simulink library "lib_primitives"  (R2026a)
settings: Solver=VariableStepAuto
undefined symbols (not defined in the file or in its folder): Cfi, fref, iC, invL, iR, iTf, L_out, omegab, R_out, Rcf
settings Model: Creator=atomas  LastModifiedBy=atomas

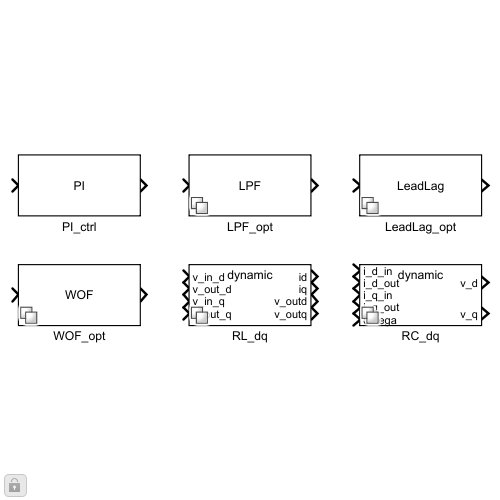
[thumbnail: Simulink's stored preview of the top-level diagram]
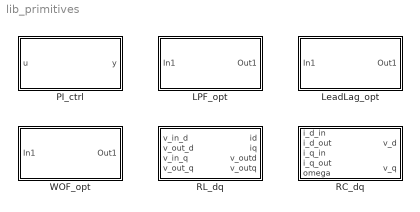
== system lib_primitives ==
  LPF_opt : Subsystem  Variant=on  mask(VFlexP_LPF_opt){T=0.01, x0=0}
      mask prompts: T "Time constant T (0=bypass)"; x0 "Initial state x0"
      mask init:
      | [iTf, use_Tf] = mask_init_opt_filter(T);
      mask Display: disp('LPF')
  LeadLag_opt : Subsystem  Variant=on  mask(VFlexP_LeadLag_opt){Tnum=1, Tden=1, x0=0}
      mask prompts: Tnum "Lead time Tnum"; Tden "Lag time Tden (0=bypass)"; x0 "Initial state x0"
      mask init:
      | [iTf, use_Tf] = mask_init_opt_filter(Tden);
      mask Display: disp('LeadLag')
  PI_ctrl : Subsystem  mask(VFlexP_PI){Kp=1, Ki=1, x0=0}
      mask prompts: Kp "Proportional gain Kp"; Ki "Integral gain Ki"; x0 "Initial condition x0"
      mask Display: disp('PI')
  RC_dq : Subsystem  Variant=on  mask{dynamic=Dynamic, R=Rcf, C=Cfi, fbase=50, x0_d=0, x0_q=0}
      mask prompts: dynamic "Dynamic behavior"; R "Parallel resistance (p.u.)"; C "Capacitance (p.u.)"; fbase "Base frequency (Hz)"; x0_d "Initial v_d"; x0_q "Initial v_q"
      mask init:
      | [iC, iR, omegab, rc_mode] = mask_init_RC(dynamic, R, C, fbase);
      mask TypeOptions dynamic: Dynamic | Static | Static omega
  RL_dq : Subsystem  Variant=on  mask{dynamic=Dynamic, R=R_out, L=L_out, fbase=50, x0_d=0, x0_q=0}
      mask prompts: dynamic "Dynamic behavior"; R "Series resistance (p.u.)"; L "Inductance (p.u.)"; fbase "Base frequency (Hz)"; x0_d "Initial i_d"; x0_q "Initial i_q"
      mask init:
      | [invL, omegab, rl_mode] = mask_init_RL(dynamic, L, fbase);
      mask TypeOptions dynamic: Static | Dynamic | Static omega
  WOF_opt : Subsystem  Variant=on  mask(VFlexP_WOF_opt){K=1, T=1, x0=0}
      mask prompts: K "Gain K"; T "Washout T (0=bypass)"; x0 "Initial state x0"
      mask init:
      | [iTf, use_Tf] = mask_init_opt_filter(T); if all(K == 0), use_Tf = 0; end
      mask Display: disp('WOF')

== system lib_primitives/LPF_opt ==
  note: 1) Add Subsystem or Model blocks as valid variant choices.
      | 2) You cannot connect blocks at this level. At simulation, connectivity is automatically
      | determined, based on the active variant and port name matching.
  In1 : Inport
  Active : Subsystem  VariantControl=use_Tf == 1
  Bypass : Subsystem  VariantControl=(default)
  Out1 : Outport

== system lib_primitives/LeadLag_opt ==
  note: 1) Add Subsystem or Model blocks as valid variant choices.
      | 2) You cannot connect blocks at this level. At simulation, connectivity is automatically
      | determined, based on the active variant and port name matching.
  In1 : Inport
  Active : Subsystem  VariantControl=use_Tf == 1
  Bypass : Subsystem  VariantControl=(default)
  Out1 : Outport

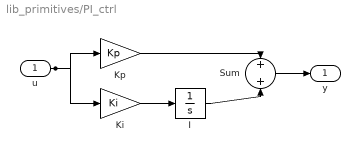
== system lib_primitives/PI_ctrl ==
  u : Inport
  I : Integrator  InitialCondition=x0
  Ki : Gain  Gain=Ki
  Kp : Gain  Gain=Kp
  Sum : Sum
  y : Outport
  wires:
  u/1 -> Kp/1, Ki/1
  Kp/1 -> Sum/1
  Ki/1 -> I/1
  I/1 -> Sum/2
  Sum/1 -> y/1

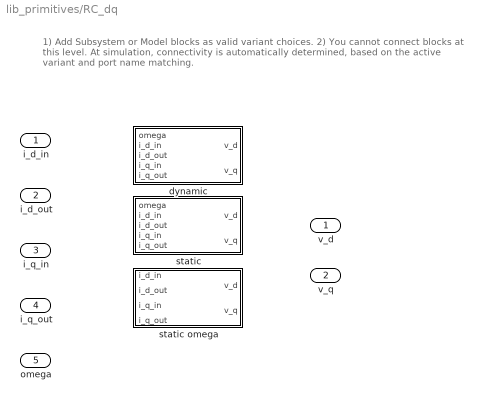
== system lib_primitives/RC_dq ==
  note: 1) Add Subsystem or Model blocks as valid variant choices.
      | 2) You cannot connect blocks at this level. At simulation, connectivity is automatically
      | determined, based on the active variant and port name matching.
  i_d_in : Inport
  i_d_out : Inport  Port=2
  i_q_in : Inport  Port=3
  i_q_out : Inport  Port=4
  omega : Inport  Port=5
  dynamic : Subsystem  VariantControl=rc_mode == 1  mask{v_d_0=1}
      mask prompts: v_d_0 "Initial condition for v_d"
  static : Subsystem  VariantControl=rc_mode == 2
  static omega : Subsystem  VariantControl=(default)
  v_d : Outport
  v_q : Outport  Port=2

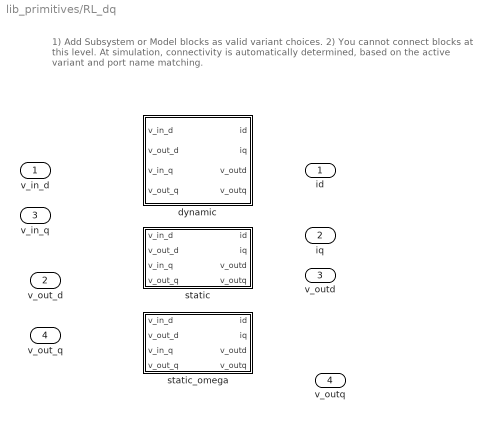
== system lib_primitives/RL_dq ==
  note: 1) Add Subsystem or Model blocks as valid variant choices.
      | 2) You cannot connect blocks at this level. At simulation, connectivity is automatically
      | determined, based on the active variant and port name matching.
  v_in_d : Inport
  v_out_d : Inport  Port=2
  v_in_q : Inport  Port=3
  v_out_q : Inport  Port=4
  dynamic : Subsystem  VariantControl=rl_mode == 1
  static : Subsystem  VariantControl=rl_mode == 2
  static_omega : Subsystem  VariantControl=(default)
  id : Outport
  iq : Outport  Port=2
  v_outd : Outport  Port=3
  v_outq : Outport  Port=4

== system lib_primitives/WOF_opt ==
  note: 1) Add Subsystem or Model blocks as valid variant choices.
      | 2) You cannot connect blocks at this level. At simulation, connectivity is automatically
      | determined, based on the active variant and port name matching.
  In1 : Inport
  Active : Subsystem  VariantControl=use_Tf == 1
  Bypass : Subsystem  VariantControl=(default)
  Out1 : Outport

== system lib_primitives/LPF_opt/Active ==
  In1 : Inport
  I : Integrator  InitialCondition=x0
  Sum : Sum  Inputs=+-
  iTf : Gain  Gain=iTf
  Out1 : Outport
  wires:
  In1/1 -> Sum/1
  Sum/1 -> iTf/1
  iTf/1 -> I/1
  I/1 -> Out1/1, Sum/2

== system lib_primitives/LPF_opt/Bypass ==
  In1 : Inport
  Out1 : Outport
  wires:
  In1/1 -> Out1/1

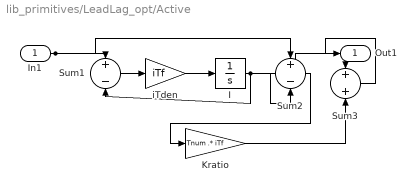
== system lib_primitives/LeadLag_opt/Active ==
  In1 : Inport
  I : Integrator  InitialCondition=x0
  Kratio : Gain  Gain=Tnum .* iTf
  Sum1 : Sum  Inputs=+-
  Sum2 : Sum  Inputs=+-
  Sum3 : Sum
  iTden : Gain  Gain=iTf
  Out1 : Outport
  wires:
  In1/1 -> Sum1/1, Sum2/1
  Sum1/1 -> iTden/1
  iTden/1 -> I/1
  I/1 -> Sum1/2, Sum2/2, Sum3/1
  Sum2/1 -> Kratio/1
  Kratio/1 -> Sum3/2
  Sum3/1 -> Out1/1

== system lib_primitives/LeadLag_opt/Bypass ==
  In1 : Inport
  Out1 : Outport
  wires:
  In1/1 -> Out1/1

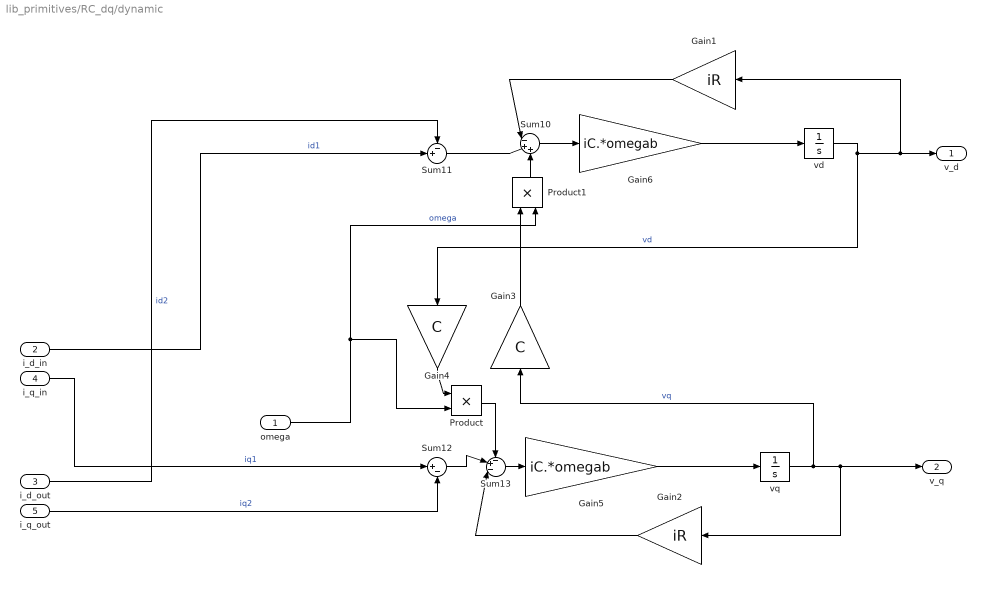
== system lib_primitives/RC_dq/dynamic ==
  omega : Inport
  i_d_in : Inport  Port=2
  i_d_out : Inport  Port=3
  i_q_in : Inport  Port=4
  i_q_out : Inport  Port=5
  Gain1 : Gain  Gain=iR
  Gain2 : Gain  Gain=iR
  Gain3 : Gain  Gain=C
  Gain4 : Gain  Gain=C
  Gain5 : Gain  Gain=iC.*omegab
  Gain6 : Gain  Gain=iC.*omegab
  Product : Product
  Product1 : Product
  Sum10 : Sum  Inputs=|-++
  Sum11 : Sum  Inputs=-+|
  Sum12 : Sum  Inputs=|+-
  Sum13 : Sum  Inputs=-+-|
  vd : Integrator  InitialCondition=x0_d
  vq : Integrator  InitialCondition=x0_q
  v_d : Outport
  v_q : Outport  Port=2
  wires:
  Sum10/1 -> Gain6/1
  Gain3/1 -> Product1/1
  vq/1 -> v_q/1, Gain2/1, Gain3/1  "vq"
  Product1/1 -> Sum10/3
  Gain4/1 -> Product/1
  Gain2/1 -> Sum13/3
  Product/1 -> Sum13/1
  Sum11/1 -> Sum10/2
  Gain6/1 -> vd/1
  omega/1 -> Product/2, Product1/2  "omega"
  Sum13/1 -> Gain5/1
  Gain1/1 -> Sum10/1
  Gain5/1 -> vq/1
  Sum12/1 -> Sum13/2
  vd/1 -> Gain4/1, v_d/1, Gain1/1  "vd"
  i_d_in/1 -> Sum11/2  "id1"
  i_d_out/1 -> Sum11/1  "id2"
  i_q_in/1 -> Sum12/1  "iq1"
  i_q_out/1 -> Sum12/2  "iq2"

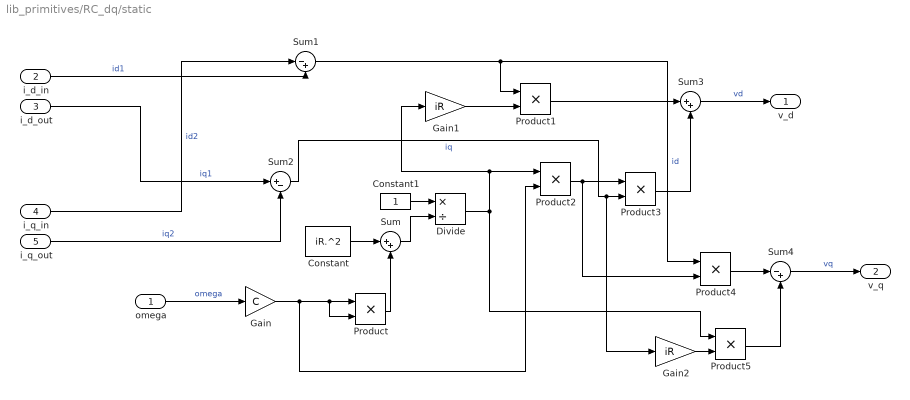
== system lib_primitives/RC_dq/static ==
  omega : Inport
  i_d_in : Inport  Port=2
  i_d_out : Inport  Port=3
  i_q_in : Inport  Port=4
  i_q_out : Inport  Port=5
  Constant : Constant  Value=iR.^2
  Constant1 : Constant
  Divide : Product  Inputs=*/
  Gain : Gain  Gain=C
  Gain1 : Gain  Gain=iR
  Gain2 : Gain  Gain=iR
  Product{,1..5} (6 alike) : Product
  Sum : Sum  Inputs=|++
  Sum1 : Sum  Inputs=|-+
  Sum2 : Sum  Inputs=|+-
  Sum3 : Sum  Inputs=|++
  Sum4 : Sum  Inputs=|-+
  v_d : Outport
  v_q : Outport  Port=2
  wires:
  Product5/1 -> Sum4/2
  Gain2/1 -> Product5/2
  Product4/1 -> Sum4/1
  Product2/1 -> Product3/1, Product4/2
  Product3/1 -> Sum3/2
  Product1/1 -> Sum3/1
  Divide/1 -> Product2/1, Gain1/1, Product5/1
  Gain1/1 -> Product1/2
  Sum2/1 -> Product3/2, Gain2/1  "iq"
  Sum1/1 -> Product4/1, Product1/1  "id"
  Constant1/1 -> Divide/1
  Product/1 -> Sum/2
  Gain/1 -> Product/1, Product/2, Product2/2
  Sum/1 -> Divide/2
  Constant/1 -> Sum/1
  Sum4/1 -> v_q/1  "vq"
  Sum3/1 -> v_d/1  "vd"
  omega/1 -> Gain/1  "omega"
  i_d_in/1 -> Sum1/2  "id1"
  i_q_in/1 -> Sum1/1  "id2"
  i_d_out/1 -> Sum2/1  "iq1"
  i_q_out/1 -> Sum2/2  "iq2"

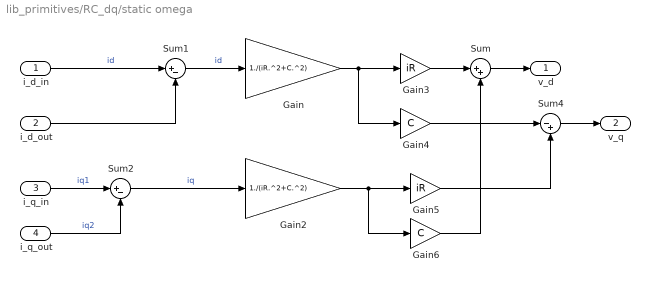
== system lib_primitives/RC_dq/static omega ==
  i_d_in : Inport
  i_d_out : Inport  Port=2
  i_q_in : Inport  Port=3
  i_q_out : Inport  Port=4
  Gain : Gain  Gain=1./(iR.^2+C.^2)
  Gain2 : Gain  Gain=1./(iR.^2+C.^2)
  Gain3 : Gain  Gain=iR
  Gain4 : Gain  Gain=C
  Gain5 : Gain  Gain=iR
  Gain6 : Gain  Gain=C
  Sum : Sum  Inputs=|++
  Sum1 : Sum  Inputs=|+-
  Sum2 : Sum  Inputs=|+-
  Sum4 : Sum  Inputs=|-+
  v_d : Outport
  v_q : Outport  Port=2
  wires:
  i_q_in/1 -> Sum2/1  "iq1"
  Sum1/1 -> Gain/1  "id"
  Sum2/1 -> Gain2/1  "iq"
  i_q_out/1 -> Sum2/2  "iq2"
  i_d_in/1 -> Sum1/1  "id"
  i_d_out/1 -> Sum1/2
  Gain/1 -> Gain4/1, Gain3/1
  Gain2/1 -> Gain6/1, Gain5/1
  Gain3/1 -> Sum/1
  Gain6/1 -> Sum/2
  Gain4/1 -> Sum4/1
  Gain5/1 -> Sum4/2
  Sum4/1 -> v_q/1
  Sum/1 -> v_d/1

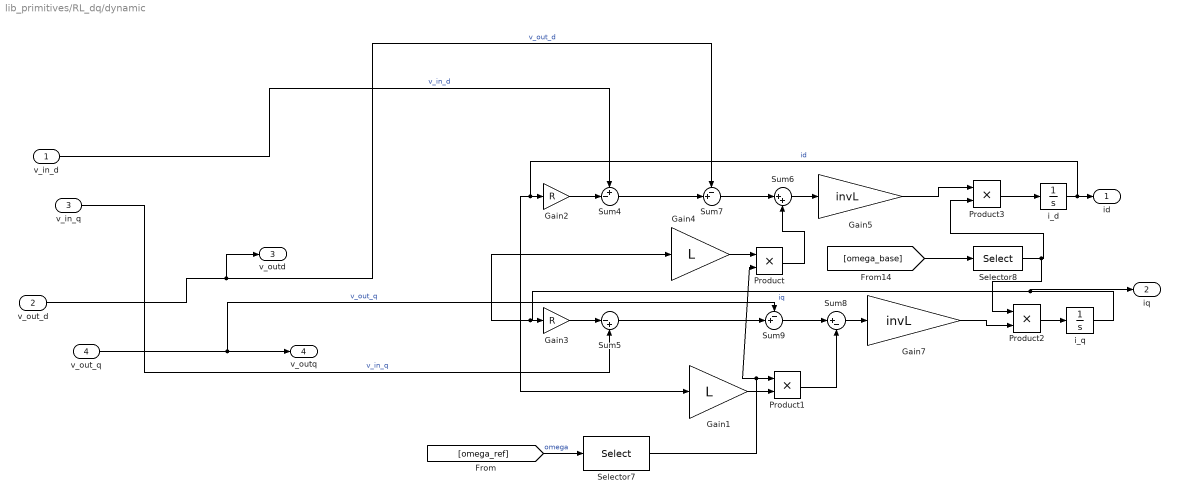
== system lib_primitives/RL_dq/dynamic ==
  v_in_d : Inport
  v_out_d : Inport  Port=2
  v_in_q : Inport  Port=3
  v_out_q : Inport  Port=4
  Gain1 : Gain  Gain=L
  Gain2 : Gain  Gain=R
  Gain3 : Gain  Gain=R
  Gain4 : Gain  Gain=L
  Gain5 : Gain  Gain=invL
  Gain7 : Gain  Gain=invL
  Product{,1..3} (4 alike) : Product
  Selector7 : Selector  InputPortWidth=length(fref.ref_units)  IndexOptions=Index vector (dialog)  Indices=block_fref  OutputSizes=1
  Selector8 : Selector  InputPortWidth=length(fref.ref_units)  IndexOptions=Index vector (dialog)  Indices=block_fref  OutputSizes=1
  Sum4 : Sum  Inputs=+-|
  Sum5 : Sum  Inputs=|-+
  Sum6 : Sum  Inputs=|++
  Sum7 : Sum  Inputs=-+|
  Sum8 : Sum  Inputs=|+-
  Sum9 : Sum  Inputs=-+|
  i_d : Integrator  InitialCondition=x0_d
  i_q : Integrator  InitialCondition=x0_q
  id : Outport
  iq : Outport  Port=2
  v_outd : Outport  Port=3
  v_outq : Outport  Port=4
  wires:
  Gain7/1 -> Product2/2
  Product2/1 -> i_q/1
  Gain5/1 -> Product3/1
  Product3/1 -> i_d/1
  Selector8/1 -> Product3/2, Product2/1
  [omega_base] -> Selector8/1
  Selector7/1 -> Product/2, Product1/1
  v_out_q/1 -> v_outq/1, Sum9/1  "v_out_q"
  v_out_d/1 -> v_outd/1, Sum7/1  "v_out_d"
  Sum9/1 -> Sum8/1
  Gain1/1 -> Product1/2
  i_q/1 -> iq/1, Gain4/1, Gain3/1  "iq"
  Sum5/1 -> Sum9/2
  Gain3/1 -> Sum5/1
  Sum7/1 -> Sum6/1
  Gain4/1 -> Product/1
  Product1/1 -> Sum8/2
  Sum4/1 -> Sum7/2
  Sum8/1 -> Gain7/1
  Product/1 -> Sum6/2
  [omega_ref] -> Selector7/1  "omega"
  Sum6/1 -> Gain5/1
  i_d/1 -> Gain2/1, Gain1/1, id/1  "id"
  Gain2/1 -> Sum4/2
  v_in_d/1 -> Sum4/1  "v_in_d"
  v_in_q/1 -> Sum5/2  "v_in_q"

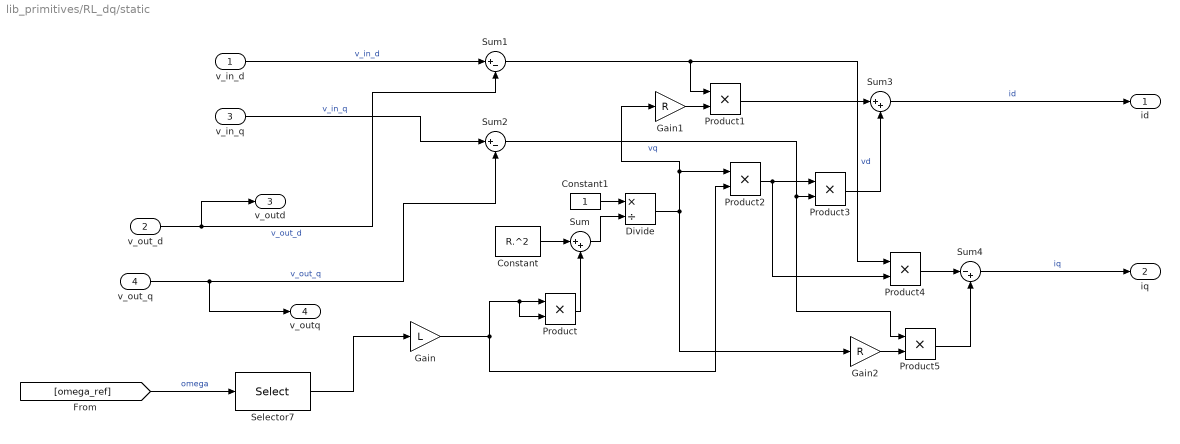
== system lib_primitives/RL_dq/static ==
  v_in_d : Inport
  v_out_d : Inport  Port=2
  v_in_q : Inport  Port=3
  v_out_q : Inport  Port=4
  Constant : Constant  Value=R.^2
  Constant1 : Constant
  Divide : Product  Inputs=*/
  Gain : Gain  Gain=L
  Gain1 : Gain  Gain=R
  Gain2 : Gain  Gain=R
  Product{,1..5} (6 alike) : Product
  Selector7 : Selector  InputPortWidth=length(fref.ref_units)  IndexOptions=Index vector (dialog)  Indices=block_fref  OutputSizes=1
  Sum : Sum  Inputs=|++
  Sum1 : Sum  Inputs=|+-
  Sum2 : Sum  Inputs=|+-
  Sum3 : Sum  Inputs=|++
  Sum4 : Sum  Inputs=|-+
  id : Outport
  iq : Outport  Port=2
  v_outd : Outport  Port=3
  v_outq : Outport  Port=4
  wires:
  Selector7/1 -> Gain/1
  [omega_ref] -> Selector7/1  "omega"
  v_in_d/1 -> Sum1/1  "v_in_d"
  v_out_q/1 -> v_outq/1, Sum2/2  "v_out_q"
  Sum4/1 -> iq/1  "iq"
  Sum3/1 -> id/1  "id"
  Gain1/1 -> Product1/2
  Product2/1 -> Product4/2, Product3/1
  Product4/1 -> Sum4/1
  Divide/1 -> Gain2/1, Gain1/1, Product2/1
  Sum1/1 -> Product1/1, Product4/1  "vd"
  Product3/1 -> Sum3/2
  Constant1/1 -> Divide/1
  Gain/1 -> Product/2, Product/1, Product2/2
  Sum2/1 -> Product5/1, Product3/2  "vq"
  Constant/1 -> Sum/1
  Product5/1 -> Sum4/2
  Product1/1 -> Sum3/1
  Product/1 -> Sum/2
  Gain2/1 -> Product5/2
  Sum/1 -> Divide/2
  v_out_d/1 -> v_outd/1, Sum1/2  "v_out_d"
  v_in_q/1 -> Sum2/1  "v_in_q"

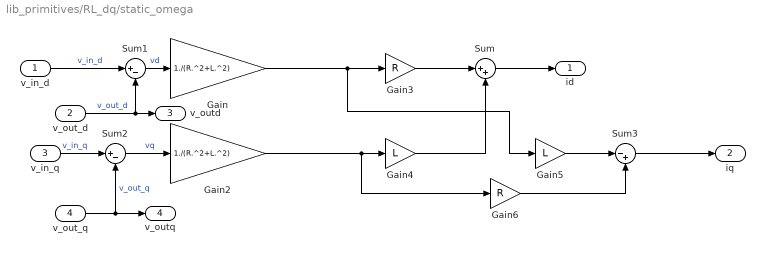
== system lib_primitives/RL_dq/static_omega ==
  v_in_d : Inport
  v_out_d : Inport  Port=2
  v_in_q : Inport  Port=3
  v_out_q : Inport  Port=4
  Gain : Gain  Gain=1./(R.^2+L.^2)
  Gain2 : Gain  Gain=1./(R.^2+L.^2)
  Gain3 : Gain  Gain=R
  Gain4 : Gain  Gain=L
  Gain5 : Gain  Gain=L
  Gain6 : Gain  Gain=R
  Sum : Sum  Inputs=|++
  Sum1 : Sum  Inputs=|+-
  Sum2 : Sum  Inputs=|+-
  Sum3 : Sum  Inputs=|-+
  id : Outport
  iq : Outport  Port=2
  v_outd : Outport  Port=3
  v_outq : Outport  Port=4
  wires:
  v_in_q/1 -> Sum2/1  "v_in_q"
  v_in_d/1 -> Sum1/1  "v_in_d"
  v_out_q/1 -> v_outq/1, Sum2/2  "v_out_q"
  v_out_d/1 -> v_outd/1, Sum1/2  "v_out_d"
  Sum1/1 -> Gain/1  "vd"
  Sum2/1 -> Gain2/1  "vq"
  Gain/1 -> Gain5/1, Gain3/1
  Gain3/1 -> Sum/1
  Gain4/1 -> Sum/2
  Gain2/1 -> Gain6/1, Gain4/1
  Sum/1 -> id/1
  Gain5/1 -> Sum3/1
  Sum3/1 -> iq/1
  Gain6/1 -> Sum3/2

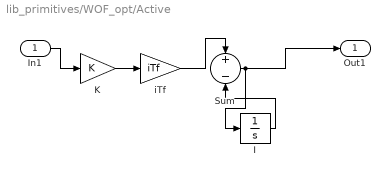
== system lib_primitives/WOF_opt/Active ==
  In1 : Inport
  I : Integrator  InitialCondition=x0
  K : Gain  Gain=K
  Sum : Sum  Inputs=+-
  iTf : Gain  Gain=iTf
  Out1 : Outport
  wires:
  In1/1 -> K/1
  K/1 -> iTf/1
  iTf/1 -> Sum/1
  I/1 -> Sum/2
  Sum/1 -> I/1, Out1/1

== system lib_primitives/WOF_opt/Bypass ==
  In1 : Inport
  Zero : Gain  Gain=0
  Out1 : Outport
  wires:
  In1/1 -> Zero/1
  Zero/1 -> Out1/1
